simulink subsystem "LEDs"  (R2022b)
settings: Solver=VariableStepAuto  StartTime=0.0  StopTime=10.0  RelTol=1e-3
libraries: simulink x4, arduinolib x3
settings Model: Creator=miriamfreiriasanjuan  LastModifiedBy=miriamfreiriasanjuan

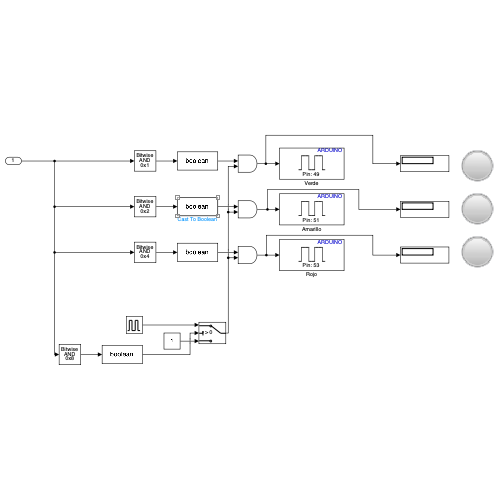
[thumbnail: Simulink's stored preview of the top-level diagram]
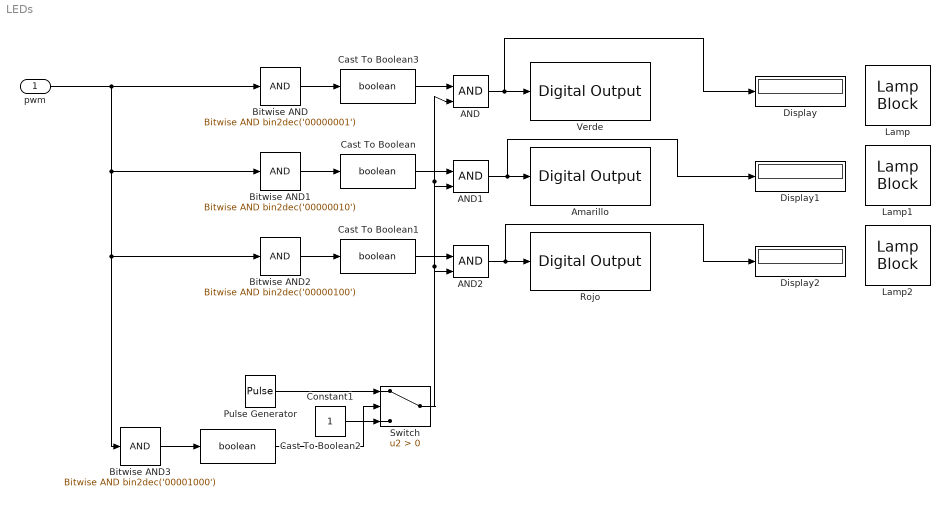
== system LEDs ==
  pwm : Inport
  AND : Logic  IconShape=distinctive  AllPortsSameDT=off  OutDataTypeStr=boolean
  AND1 : Logic  IconShape=distinctive  AllPortsSameDT=off  OutDataTypeStr=boolean
  AND2 : Logic  IconShape=distinctive  AllPortsSameDT=off  OutDataTypeStr=boolean
  Amarillo : arduinolib/Digital Output  pinNumber=51  Direction=output  blockPlatform=arduino
  Bitwise AND : simulink/Logic and Bit Operations/Bitwise Operator  logicop=AND  UseBitMask=on  BitMask=bin2dec('00000001')  BitMaskRealWorld=Stored Integer
      settings: LibrarySourceBlock=|
      | simulink/Quick Insert/Logic and Bit
      | Operations/Bitwise AND
  Bitwise AND1 : simulink/Logic and Bit Operations/Bitwise Operator  logicop=AND  UseBitMask=on  BitMask=bin2dec('00000010')  BitMaskRealWorld=Stored Integer
      settings: LibrarySourceBlock=|
      | simulink/Quick Insert/Logic and Bit
      | Operations/Bitwise AND
  Bitwise AND2 : simulink/Logic and Bit Operations/Bitwise Operator  logicop=AND  UseBitMask=on  BitMask=bin2dec('00000100')  BitMaskRealWorld=Stored Integer
      settings: LibrarySourceBlock=|
      | simulink/Quick Insert/Logic and Bit
      | Operations/Bitwise AND
  Bitwise AND3 : simulink/Logic and Bit Operations/Bitwise Operator  logicop=AND  UseBitMask=on  BitMask=bin2dec('00001000')  BitMaskRealWorld=Stored Integer
      settings: LibrarySourceBlock=|
      | simulink/Quick Insert/Logic and Bit
      | Operations/Bitwise AND
  Cast To Boolean{,1..3} (4 alike) : DataTypeConversion  OutDataTypeStr=boolean  SaturateOnIntegerOverflow=off  RndMeth=Floor
  Constant1 : Constant
  Display : Display
  Display1 : Display
  Display2 : Display
  Lamp : LampBlock  LabelPosition=Hide
  Lamp1 : LampBlock  LabelPosition=Hide
  Lamp2 : LampBlock  LabelPosition=Hide
  Pulse Generator : DiscretePulseGenerator  PulseType=Time based  Period=0.5  PulseWidth=50
  Rojo : arduinolib/Digital Output  pinNumber=53  Direction=output  blockPlatform=arduino
  Switch : Switch  Criteria=u2 > Threshold  SaturateOnIntegerOverflow=off  InputSameDT=off
  Verde : arduinolib/Digital Output  pinNumber=49  Direction=output  blockPlatform=arduino
  wires:
  Pulse Generator/1 -> Switch/1
  Cast To Boolean2/1 -> Switch/2
  Switch/1 -> AND2/2, AND1/2, AND/2
  AND2/1 -> Display2/1, Rojo/1
  Bitwise AND/1 -> Cast To Boolean3/1
  pwm/1 -> Bitwise AND1/1, Bitwise AND3/1, Bitwise AND2/1, Bitwise AND/1
  AND1/1 -> Display1/1, Amarillo/1
  Constant1/1 -> Switch/3
  Cast To Boolean/1 -> AND1/1
  Bitwise AND3/1 -> Cast To Boolean2/1
  Cast To Boolean1/1 -> AND2/1
  AND/1 -> Display/1, Verde/1
  Bitwise AND1/1 -> Cast To Boolean/1
  Bitwise AND2/1 -> Cast To Boolean1/1
  Cast To Boolean3/1 -> AND/1
